simulink model "im_inv_sensorless_ctrl_model"  (R2026a)
settings: Solver=ode1  StopTime=simlength  FixedStep=tc  MaxStep=tc  EnableMultiTasking=on
values from neighbouring files (symbols this model uses):
  cp = 2    [im_param_calc_3.m]
  Ibez = Inom*sqrt(2)    [im_param_calc_3.m]
  Lm = Ls - Lds    [im_param_calc_3.m]
  Lr = Lm + Ldr    [im_param_calc_3.m]
  Ls = Vnom/sqrt(3)/I0/(2*pi*fnom)    [im_param_calc_3.m]
  Rr = Rr+deltaRr    (= 0.00099)    [im_param_calc_3.m]
  Rs = PhaseResistance    (= 0.009)    [im_param_calc_3.m]
undefined symbols (not defined in the file or in its folder): Adrso_im, alpha_norm, beta_norm, Crso_im, CTRPIFF_CLIP_RELEASE, dead_time, DiscIntNeverNeededParam, emf_fb_p, emf_p, fi_rot_ref_norm, fPWM_INV, gamma_norm, iq_lim, Jm_model, kg, ki_inv_d, ki_inv_q, ki_w, kp_inv_d, kp_inv_q, kp_w, kw, Ldrso_im, Lm_norm, Lr_norm, Ls_norm, magnitude, Omega_r_bez, Omega_s_bez, Rs_norm, sigma_norm, simlength, tc, Tcontrol_INV, timeRamp, Tload, ts_afe, ts_inv, uf_omega_ref, uf_uq_ref, wref
libraries: nesl_utility x64, fl_lib x49, simulink x2, im_uvw_2_lib x1, threephase_inductor_lib x1, cstblocks_lti x1
(part 4 of 4)

== system im_inv_sensorless_ctrl_model/inverter//ctrl/inverter/inverter/sv_pwm/modulator1/PWM generator 3 ==
  m_index : Inport
  phase : Inport  Port=2
  Clock : Clock
  Constant : Constant  Value=dead_time*f
  Constant1 : Constant  Value=polarity
  Constant2 : Constant  Value=1/f
  Constant4 : Constant
  Data Type Conversion1 : DataTypeConversion
  Data Type Conversion2 : DataTypeConversion
  Gain4 : Gain  Gain=1/2
  Gain5 : Gain  Gain=1/(pi/2)
  Hit Crossing : HitCross  ShowOutputPort=off
  Hit Crossing1 : HitCross  ShowOutputPort=off
  MATLAB Function : MATLAB Function  TreatAsAtomicUnit=on
  Relational Operator1 : RelationalOperator  Operator=<=  InputSameDT=off
  Relational Operator2 : RelationalOperator  Operator=<=  InputSameDT=off
  Relay : Relay  OnOutputValue=pos_cmd_gate  OffOutputValue=neg_cmd_gate
  Relay1 : Relay  OnOutputValue=pos_cmd_gate  OffOutputValue=neg_cmd_gate
  Saturation1 : Saturate  UpperLimit=m_up  LowerLimit=m_low
  Sum : Sum  Inputs=|++  SaturateOnIntegerOverflow=on
  Sum1 : Sum  Inputs=-+|  SaturateOnIntegerOverflow=on
  Sum3 : Sum  Inputs=|++
  Switch : Switch  Criteria=u2 > Threshold  SaturateOnIntegerOverflow=off  InputSameDT=off
  Switch1 : Switch  Criteria=u2 > Threshold  SaturateOnIntegerOverflow=off  InputSameDT=off
  m1 : Outport
  m2 : Outport  Port=2
  wires:
  Relational Operator1/1 -> Data Type Conversion1/1
  m_index/1 -> Saturation1/1
  Relational Operator2/1 -> Data Type Conversion2/1
  Data Type Conversion2/1 -> Switch/1, Switch1/3, Hit Crossing1/1
  Constant/1 -> Sum/2, Sum1/1
  Saturation1/1 -> Sum/1, Sum1/2
  Sum/1 -> Relational Operator1/1
  Sum1/1 -> Relational Operator2/2
  Gain4/1 -> Relational Operator2/1, Relational Operator1/2
  Data Type Conversion1/1 -> Hit Crossing/1, Switch/3, Switch1/1
  Switch/1 -> Relay/1
  Clock/1 -> MATLAB Function/1(t)
  Constant2/1 -> MATLAB Function/3(period)
  phase/1 -> MATLAB Function/2(phase)
  MATLAB Function/1(y) -> Gain5/1
  Gain5/1 -> Sum3/1
  Sum3/1 -> Gain4/1
  Constant4/1 -> Sum3/2
  Relay/1 -> m2/1
  Constant1/1 -> Switch1/2, Switch/2
  Switch1/1 -> Relay1/1
  Relay1/1 -> m1/1

== system im_inv_sensorless_ctrl_model/inverter//ctrl/inverter/inverter/three phase pwm/modulator/PWM generator 1 ==
  m_index : Inport
  phase : Inport  Port=2
  Clock : Clock
  Constant : Constant  Value=dead_time*f
  Constant2 : Constant  Value=1/f
  Constant4 : Constant
  Data Type Conversion1 : DataTypeConversion
  Data Type Conversion2 : DataTypeConversion
  Gain2 : Gain  Gain=vg_firing
  Gain3 : Gain  Gain=vg_firing
  Gain4 : Gain  Gain=1/2
  Gain5 : Gain  Gain=1/(pi/2)
  Hit Crossing : HitCross  ShowOutputPort=off
  Hit Crossing1 : HitCross  ShowOutputPort=off
  MATLAB Function : MATLAB Function  TreatAsAtomicUnit=on
  Relational Operator1 : RelationalOperator  Operator=<=  InputSameDT=off
  Relational Operator2 : RelationalOperator  Operator=<=  InputSameDT=off
  Saturation1 : Saturate  UpperLimit=m_up  LowerLimit=m_low
  Sum : Sum  Inputs=|++  SaturateOnIntegerOverflow=on
  Sum1 : Sum  Inputs=-+|  SaturateOnIntegerOverflow=on
  Sum3 : Sum  Inputs=|++
  m1 : Outport
  m2 : Outport  Port=2
  wires:
  Relational Operator1/1 -> Data Type Conversion1/1
  m_index/1 -> Saturation1/1
  Relational Operator2/1 -> Data Type Conversion2/1
  Data Type Conversion2/1 -> Gain3/1, Hit Crossing1/1
  Constant/1 -> Sum/2, Sum1/1
  Saturation1/1 -> Sum/1, Sum1/2
  Sum/1 -> Relational Operator1/1
  Sum1/1 -> Relational Operator2/2
  Gain4/1 -> Relational Operator2/1, Relational Operator1/2
  Data Type Conversion1/1 -> Hit Crossing/1, Gain2/1
  Gain2/1 -> m1/1
  Gain3/1 -> m2/1
  Clock/1 -> MATLAB Function/1(t)
  Constant2/1 -> MATLAB Function/3(period)
  phase/1 -> MATLAB Function/2(phase)
  MATLAB Function/1(y) -> Gain5/1
  Gain5/1 -> Sum3/1
  Sum3/1 -> Gain4/1
  Constant4/1 -> Sum3/2

== system im_inv_sensorless_ctrl_model/inverter//ctrl/inverter/inverter/three phase pwm/modulator/PWM generator 2 ==
  m_index : Inport
  phase : Inport  Port=2
  Clock : Clock
  Constant : Constant  Value=dead_time*f
  Constant2 : Constant  Value=1/f
  Constant4 : Constant
  Data Type Conversion1 : DataTypeConversion
  Data Type Conversion2 : DataTypeConversion
  Gain2 : Gain  Gain=vg_firing
  Gain3 : Gain  Gain=vg_firing
  Gain4 : Gain  Gain=1/2
  Gain5 : Gain  Gain=1/(pi/2)
  Hit Crossing : HitCross  ShowOutputPort=off
  Hit Crossing1 : HitCross  ShowOutputPort=off
  MATLAB Function : MATLAB Function  TreatAsAtomicUnit=on
  Relational Operator1 : RelationalOperator  Operator=<=  InputSameDT=off
  Relational Operator2 : RelationalOperator  Operator=<=  InputSameDT=off
  Saturation1 : Saturate  UpperLimit=m_up  LowerLimit=m_low
  Sum : Sum  Inputs=|++  SaturateOnIntegerOverflow=on
  Sum1 : Sum  Inputs=-+|  SaturateOnIntegerOverflow=on
  Sum3 : Sum  Inputs=|++
  m1 : Outport
  m2 : Outport  Port=2
  wires:
  Constant4/1 -> Sum3/2
  Sum3/1 -> Gain4/1
  Gain5/1 -> Sum3/1
  MATLAB Function/1(y) -> Gain5/1
  phase/1 -> MATLAB Function/2(phase)
  Constant2/1 -> MATLAB Function/3(period)
  Clock/1 -> MATLAB Function/1(t)
  Gain3/1 -> m2/1
  Gain2/1 -> m1/1
  Data Type Conversion1/1 -> Gain2/1, Hit Crossing/1
  Gain4/1 -> Relational Operator1/2, Relational Operator2/1
  Sum1/1 -> Relational Operator2/2
  Sum/1 -> Relational Operator1/1
  Saturation1/1 -> Sum1/2, Sum/1
  Constant/1 -> Sum1/1, Sum/2
  Data Type Conversion2/1 -> Hit Crossing1/1, Gain3/1
  Relational Operator2/1 -> Data Type Conversion2/1
  m_index/1 -> Saturation1/1
  Relational Operator1/1 -> Data Type Conversion1/1

== system im_inv_sensorless_ctrl_model/inverter//ctrl/inverter/inverter/three phase pwm/modulator/PWM generator 3 ==
  m_index : Inport
  phase : Inport  Port=2
  Clock : Clock
  Constant : Constant  Value=dead_time*f
  Constant2 : Constant  Value=1/f
  Constant4 : Constant
  Data Type Conversion1 : DataTypeConversion
  Data Type Conversion2 : DataTypeConversion
  Gain2 : Gain  Gain=vg_firing
  Gain3 : Gain  Gain=vg_firing
  Gain4 : Gain  Gain=1/2
  Gain5 : Gain  Gain=1/(pi/2)
  Hit Crossing : HitCross  ShowOutputPort=off
  Hit Crossing1 : HitCross  ShowOutputPort=off
  MATLAB Function : MATLAB Function  TreatAsAtomicUnit=on
  Relational Operator1 : RelationalOperator  Operator=<=  InputSameDT=off
  Relational Operator2 : RelationalOperator  Operator=<=  InputSameDT=off
  Saturation1 : Saturate  UpperLimit=m_up  LowerLimit=m_low
  Sum : Sum  Inputs=|++  SaturateOnIntegerOverflow=on
  Sum1 : Sum  Inputs=-+|  SaturateOnIntegerOverflow=on
  Sum3 : Sum  Inputs=|++
  m1 : Outport
  m2 : Outport  Port=2
  wires:
  Relational Operator1/1 -> Data Type Conversion1/1
  m_index/1 -> Saturation1/1
  Relational Operator2/1 -> Data Type Conversion2/1
  Data Type Conversion2/1 -> Gain3/1, Hit Crossing1/1
  Constant/1 -> Sum/2, Sum1/1
  Saturation1/1 -> Sum/1, Sum1/2
  Sum/1 -> Relational Operator1/1
  Sum1/1 -> Relational Operator2/2
  Gain4/1 -> Relational Operator2/1, Relational Operator1/2
  Data Type Conversion1/1 -> Hit Crossing/1, Gain2/1
  Gain2/1 -> m1/1
  Gain3/1 -> m2/1
  Clock/1 -> MATLAB Function/1(t)
  Constant2/1 -> MATLAB Function/3(period)
  phase/1 -> MATLAB Function/2(phase)
  MATLAB Function/1(y) -> Gain5/1
  Gain5/1 -> Sum3/1
  Sum3/1 -> Gain4/1
  Constant4/1 -> Sum3/2

== matlab function im_inv_sensorless_ctrl_model/induction motor/control performance evaluation/adc2dq_s_2/alphabeta2xieta ==
  data: alpha input; d output; beta input; theta input; q output
function [d,q] = alphabeta2xieta(alpha,beta,theta)

    d  =  alpha*cos(theta) + beta*sin(theta);
    q = -alpha*sin(theta) + beta*cos(theta);

end

== matlab function im_inv_sensorless_ctrl_model/induction motor/control performance evaluation/adc2dq_slip_2/abc2alphabeta ==
  data: abc input; alpha output; beta output
function [alpha,beta] = abc2alphabeta(abc)

alpha = 2/3*(abc(1) - 1/2*abc(2) - 1/2*abc(3));
beta  = 1/sqrt(3)*(abc(2) - abc(3));

end

== matlab function im_inv_sensorless_ctrl_model/induction motor/control performance evaluation/adc2dq_slip_2/alphabeta2xieta ==
  data: alpha input; d output; beta input; theta input; q output
function [d,q] = alphabeta2xieta(alpha,beta,theta)

    d  =  alpha*cos(theta) + beta*sin(theta);
    q = -alpha*sin(theta) + beta*cos(theta);

end

== matlab function im_inv_sensorless_ctrl_model/inverter//ctrl/im_ctrl/im_control/data_analysis/double_integrator_observer_2/bounder1 ==
  data: u input; y output
function y = bounder(u)
    
    y = -pi + mod(u+3*pi,2*pi);
end

== matlab function im_inv_sensorless_ctrl_model/inverter//ctrl/im_ctrl/im_control/data_analysis/double_integrator_observer_2/bounder2 ==
  data: u input; y output
function y = bounder(u)
    
    y = -pi + mod(u+3*pi,2*pi);
end

== matlab function im_inv_sensorless_ctrl_model/inverter//ctrl/inverter/inverter/three phase pwm1/uvw2alphabeta1 ==
  data: alpha input; u output; beta input; v output; w output
function [u,v,w] = alphabeta2uvw(alpha,beta)

u  = alpha;
v  = -0.5*alpha+sqrt(3)/2*beta;
w  = -0.5*alpha-sqrt(3)/2*beta;

end

== matlab function im_inv_sensorless_ctrl_model/inverter//ctrl/im_ctrl/im_control/data_analysis/double_integrator_observer_3/bounder1 ==
  data: u input; y output
function y = bounder(u)
    
    y = -pi + mod(u+3*pi,2*pi);
end

== matlab function im_inv_sensorless_ctrl_model/inverter//ctrl/im_ctrl/im_control/data_analysis/double_integrator_observer_3/bounder2 ==
  data: u input; y output
function y = bounder(u)
    
    y = -pi + mod(u+3*pi,2*pi);
end

== matlab function im_inv_sensorless_ctrl_model/inverter//ctrl/im_ctrl/im_control/u//f control/uf_phase_generation/bounder ==
  data: u input; y output
function y = bounder(u)
    
    u = -pi + mod(u+3*pi,2*pi);
    
    y = u;
end

== matlab function im_inv_sensorless_ctrl_model/induction motor/mechanical data/double_integrator_observer_for_im/bounder1 ==
  data: u input; y output
function y = bounder(u)
    y = -pi + mod(u+3*pi,2*pi);
end

== matlab function im_inv_sensorless_ctrl_model/inverter//ctrl/im_ctrl/im_control/data_analysis/double_integrator_observer_1/bounder2 ==
  data: u input; y output
function y = bounder(u)
    
    y = -pi + mod(u+3*pi,2*pi);
end

== matlab function im_inv_sensorless_ctrl_model/induction motor/mechanical data/encoder_measure/bounder2 ==
  data: u input; y output
function y = bounder(u) 
    y = -pi + mod(u+3*pi,2*pi);
end

== matlab function im_inv_sensorless_ctrl_model/inverter//ctrl/inverter/inverter/sv_pwm/modulator1/PWM generator 2/MATLAB Function ==
  data: t input; y output; phase input; period input
function y = trgo(t,phase,period)
x = sin(2*pi/period*t - phase -pi/2);
y = asin(x);

== matlab function im_inv_sensorless_ctrl_model/inverter//ctrl/im_ctrl/im_control/flux_estimator/bounder2 ==
  data: u input; y output
function y = bounder(u)
    
    y = -pi + mod(u+3*pi,2*pi);

end

== matlab function im_inv_sensorless_ctrl_model/inverter//ctrl/im_ctrl/im_control/flux_estimator/bounder3 ==
  data: u input; y output
function y = bounder(u)
    
    y = -pi + mod(u+3*pi,2*pi);
    
end

== matlab function im_inv_sensorless_ctrl_model/inverter//ctrl/im_ctrl/im_control/data_analysis/double_integrator_observer_1/bounder1 ==
  data: u input; y output
function y = bounder(u)
    
    y = -pi + mod(u+3*pi,2*pi);
end

== matlab function im_inv_sensorless_ctrl_model/inverter//ctrl/inverter/inverter/sv_pwm/modulator1/PWM generator 3/MATLAB Function ==
  data: t input; y output; phase input; period input
function y = trgo(t,phase,period)
x = sin(2*pi/period*t - phase -pi/2);
y = asin(x);

== matlab function im_inv_sensorless_ctrl_model/inverter//ctrl/im_ctrl/rotor_speed_observer/current_flux_estimator/obs_td/MATLAB Function ==
  data: usa input; usb input; isa input; xi_a_1 output; isb input; xi_a input; xi_b input; alpha input; beta input; gamma input; sigma input; c input; Lm input; omega_r input; xi_b_1 output; omega_base input; flux_a output; flux_b output; ts input
function [xi_a_1, xi_b_1, flux_a, flux_b] = flux_obs(usa, usb, isa, isb, xi_a, xi_b, ...
    alpha, beta, gamma, sigma, c, Lm, omega_r, omega_base, ts)
 
    xi_a_1 = xi_a + ts*omega_base*(-alpha*(1+c*beta)*xi_a - omega_r*(1+c*beta)*xi_b + ...
        ((alpha*Lm + c*gamma) - alpha*c*(1 + c*beta))*isa - omega_r*c*(1 + c*beta)*isb - ...
        c/sigma*usa);

    xi_b_1 = xi_b + ts*omega_base*(-alpha*(1+c*beta)*xi_b + omega_r*(1+c*beta)*xi_a + ...
        ((alpha*Lm + c*gamma) - alpha*c*(1 + c*beta))*isb + omega_r*c*(1 + c*beta)*isa - ...
        c/sigma*usb);

    flux_a = c*isa + xi_a;
    flux_b = c*isb + xi_b;

== matlab function im_inv_sensorless_ctrl_model/inverter//ctrl/im_ctrl/rotor_speed_observer/bounder1 ==
  data: u input; y output
function y = bounder(u)
    
    y = -pi + mod(u+3*pi,2*pi);
end

== matlab function im_inv_sensorless_ctrl_model/inverter//ctrl/im_ctrl/im_control/flux_estimator/bounder1 ==
  data: u input; y output
function y = bounder(u)
    
    y = -pi + mod(u+3*pi,2*pi);
    
end

== matlab function im_inv_sensorless_ctrl_model/inverter//ctrl/inverter/inverter/sv_pwm/modulator1/PWM generator 1/MATLAB Function ==
  data: t input; y output; phase input; period input
function y = trgo(t,phase,period)
x = sin(2*pi/period*t - phase -pi/2);
y = asin(x);

== matlab function im_inv_sensorless_ctrl_model/induction motor/control performance evaluation/adc2dq_s_1/abc2alphabeta ==
  data: abc input; alpha output; beta output
function [alpha,beta] = abc2alphabeta(abc)

alpha = 2/3*(abc(1) - 1/2*abc(2) - 1/2*abc(3));
beta  = 1/sqrt(3)*(abc(2) - abc(3));

end

== matlab function im_inv_sensorless_ctrl_model/inverter//ctrl/inverter/inverter/three phase pwm/modulator/PWM generator 1/MATLAB Function ==
  data: t input; y output; phase input; period input
function y = trgo(t,phase,period)
x = sin(2*pi/period*t - phase);
y = asin(x);

== matlab function im_inv_sensorless_ctrl_model/inverter//ctrl/inverter/inverter/three phase pwm/uvw2alphabeta1 ==
  data: alpha input; u output; beta input; v output; w output
function [u,v,w] = alphabeta2uvw(alpha,beta)

u  = alpha;
v  = -0.5*alpha+sqrt(3)/2*beta;
w  = -0.5*alpha-sqrt(3)/2*beta;

end

== matlab function im_inv_sensorless_ctrl_model/induction motor/mechanical data/double_integrator_observer_for_im/bounder2 ==
  data: u input; y output
function y = bounder(u)
    y = -pi + mod(u+3*pi,2*pi);
end

== matlab function im_inv_sensorless_ctrl_model/inverter//ctrl/inverter/inverter/three phase pwm/modulator/PWM generator 2/MATLAB Function ==
  data: t input; y output; phase input; period input
function y = trgo(t,phase,period)
x = sin(2*pi/period*t - phase);
y = asin(x);

== matlab function im_inv_sensorless_ctrl_model/inverter//ctrl/inverter/inverter/three phase pwm/modulator/PWM generator 3/MATLAB Function ==
  data: t input; y output; phase input; period input
function y = trgo(t,phase,period)
x = sin(2*pi/period*t - phase);
y = asin(x);

== matlab function im_inv_sensorless_ctrl_model/induction motor/control performance evaluation/adc2dq_slip_1/abc2alphabeta ==
  data: abc input; alpha output; beta output
function [alpha,beta] = abc2alphabeta(abc)

alpha = 2/3*(abc(1) - 1/2*abc(2) - 1/2*abc(3));
beta  = 1/sqrt(3)*(abc(2) - abc(3));

end

== matlab function im_inv_sensorless_ctrl_model/induction motor/control performance evaluation/adc2dq_slip_1/alphabeta2xieta ==
  data: alpha input; d output; beta input; theta input; q output
function [d,q] = alphabeta2xieta(alpha,beta,theta)

    d  =  alpha*cos(theta) + beta*sin(theta);
    q = -alpha*sin(theta) + beta*cos(theta);

end

== matlab function im_inv_sensorless_ctrl_model/induction motor/control performance evaluation/adc2dq_s_2/abc2alphabeta ==
  data: abc input; alpha output; beta output
function [alpha,beta] = abc2alphabeta(abc)

alpha = 2/3*(abc(1) - 1/2*abc(2) - 1/2*abc(3));
beta  = 1/sqrt(3)*(abc(2) - abc(3));

end

== matlab function im_inv_sensorless_ctrl_model/induction motor/control performance evaluation/adc2dq_s_1/alphabeta2xieta ==
  data: alpha input; d output; beta input; theta input; q output
function [d,q] = alphabeta2xieta(alpha,beta,theta)

    d  =  alpha*cos(theta) + beta*sin(theta);
    q = -alpha*sin(theta) + beta*cos(theta);

end
